simulink model "scheme_L2"  (R2023a)
settings: Solver=VariableStepAuto  StartTime=0.0  StopTime=10  MaxStep=0.01  RelTol=1e-3
settings Model: Creator=mrlin  LastModifiedBy=mrlin

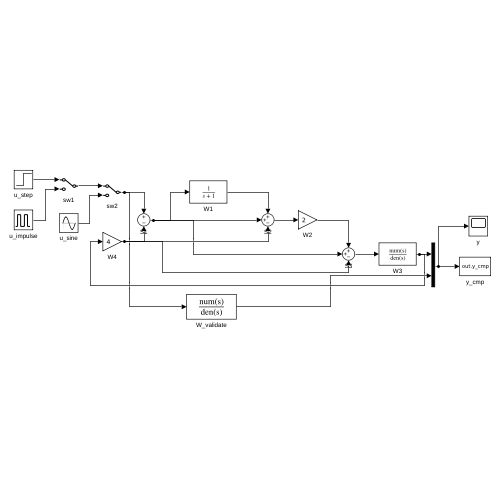
[thumbnail: Simulink's stored preview of the top-level diagram]
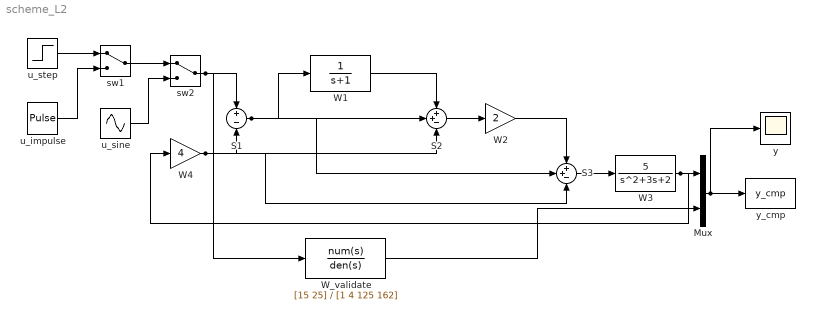
== system scheme_L2 ==
  Mux : Mux  Inputs=2
  S1 : Sum  Inputs=+-
  S2 : Sum  Inputs=++-
  S3 : Sum  Inputs=++-
  W1 : TransferFcn  Denominator=[1 1]
  W2 : Gain  Gain=2
  W3 : TransferFcn  Numerator=[5]  Denominator=[1 3 2]
  W4 : Gain  Gain=4
  W_validate : TransferFcn  Numerator=[15 25]  Denominator=[1 4 125 162]
  sw1 : ManualSwitch
  sw2 : ManualSwitch
  u_impulse : DiscretePulseGenerator  PulseType=Time based  Amplitude=100  Period=100  PulseWidth=0.01
  u_sine : Sin  SampleTime=0
  u_step : Step  Time=0  SampleTime=0
  y : Scope
  y_cmp : ToWorkspace  VariableName=y_cmp  SaveFormat=Structure With Time  SampleTime=-1
  wires:
  Mux/1 -> y/1, y_cmp/1
  u_step/1 -> sw1/1
  S3/1 -> W3/1
  u_impulse/1 -> sw1/2
  sw1/1 -> sw2/1
  W_validate/1 -> Mux/2
  u_sine/1 -> sw2/2
  W2/1 -> S3/1
  sw2/1 -> S1/1, W_validate/1
  W4/1 -> S1/2, S3/3, S2/3
  S1/1 -> W1/1, S3/2, S2/2
  W1/1 -> S2/1
  S2/1 -> W2/1
  W3/1 -> Mux/1, W4/1
